simulink library "NCR18650BD_98S45P_Library"  (R2025a)
settings: Solver=VariableStepAuto  StartTime=0.0  StopTime=10.0  RelTol=1e-3
undefined symbols (not defined in the file or in its folder): battery_builder_rtmsupport, gcbh
libraries: NCR18650BD_98S45P_Library_lib x16
(part 1 of 2)
settings Model: Creator=saarv  LastModifiedBy=saarv

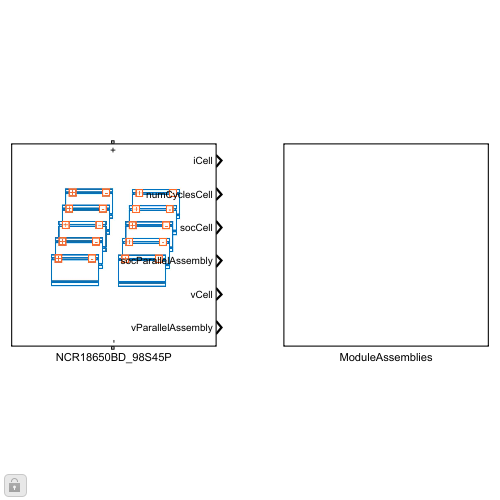
[thumbnail: Simulink's stored preview of the top-level diagram]
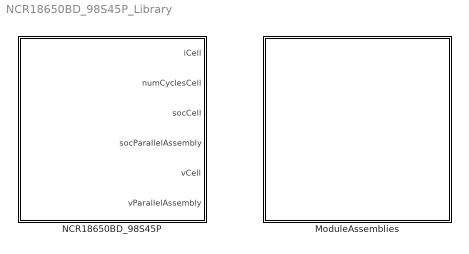
== system NCR18650BD_98S45P_Library ==
  ModuleAssemblies : Subsystem
  NCR18650BD_98S45P : Subsystem  LoadFcn=battery_builder_rtmsupport('loadfcn',gcbh);
      settings: CopyFcn=battery_builder_rtmsupport('copyfcn',gcbh);  PreCopyFcn=battery_builder_rtmsupport('precopyfcn',gcbh);  PreDeleteFcn=battery_builder_rtmsupport('predeletefcn',gcbh);  PortSchema="{\"entries\":[{\"content\":{\"sides\":[{\"content\":{\"connectorIds\":[\"LConn1\"]},\"type\":\"ConnectorPlacement.EquallySpacedRectSide\",\"uuid\":\"9e7041d5-d3d9-4996-bd95-b169094aaa75\"},{\"content\":{\"connectorIds\":[\"RConn1\"],\"side\":\"RIGHT\"},\"type\":\"ConnectorPlacement.EquallySpacedRectSide\",\"uuid\":\"1a9d726b-e110-445d-9094-f9af8985733a\"},{\"content\":{\"side\":\"TOP\"},\"type\":\"ConnectorPlacement.EquallySpacedRectSide\",\"uuid\":\"c9094138-05f6-46bf-9d7c-2f9307e18b10\"},{\"content\":{\"connectorIds\":[\"Out1\",\"Out2\",\"Out3\",\"Out4\",\"Out5\",\"Out6\"],\"side\":\"BOTTOM\"},\"type\":\"ConnectorPlacement.EquallySpacedRectSide\",\"uuid\":\"12959d5d-2702-4b18-986c-5ba3b231edc9\"}]},\"type\":\"ConnectorPlacement.EquallySpacedConnector\",\"uuid\":\"b4792a63-91de-4aa8-9329-1ac229a09e41\"}],\"packageUris\":[\"http://schema.mathworks.com/mf0/Connector/R2020b\"],\"version\":\"1.0\"}"
      mask Display: image('$imagefile')

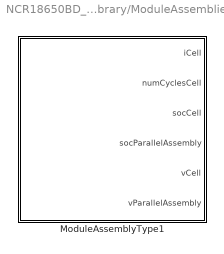
== system NCR18650BD_98S45P_Library/ModuleAssemblies ==
  ModuleAssemblyType1 : Subsystem  LoadFcn=battery_builder_rtmsupport('loadfcn',gcbh);
      settings: CopyFcn=battery_builder_rtmsupport('copyfcn',gcbh);  PreCopyFcn=battery_builder_rtmsupport('precopyfcn',gcbh);  PreDeleteFcn=battery_builder_rtmsupport('predeletefcn',gcbh);  PortSchema="{\"entries\":[{\"content\":{\"sides\":[{\"content\":{\"connectorIds\":[\"LConn1\"]},\"type\":\"ConnectorPlacement.EquallySpacedRectSide\",\"uuid\":\"9e7041d5-d3d9-4996-bd95-b169094aaa75\"},{\"content\":{\"connectorIds\":[\"RConn1\"],\"side\":\"RIGHT\"},\"type\":\"ConnectorPlacement.EquallySpacedRectSide\",\"uuid\":\"1a9d726b-e110-445d-9094-f9af8985733a\"},{\"content\":{\"side\":\"TOP\"},\"type\":\"ConnectorPlacement.EquallySpacedRectSide\",\"uuid\":\"c9094138-05f6-46bf-9d7c-2f9307e18b10\"},{\"content\":{\"connectorIds\":[\"Out1\",\"Out2\",\"Out3\",\"Out4\",\"Out5\",\"Out6\"],\"side\":\"BOTTOM\"},\"type\":\"ConnectorPlacement.EquallySpacedRectSide\",\"uuid\":\"a73cbc57-fefd-438e-a02a-7299c4782ae8\"}]},\"type\":\"ConnectorPlacement.EquallySpacedConnector\",\"uuid\":\"b4792a63-91de-4aa8-9329-1ac229a09e41\"}],\"packageUris\":[\"http://schema.mathworks.com/mf0/Connector/R2020b\"],\"version\":\"1.0\"}"
      mask Display: image('$imagefile')

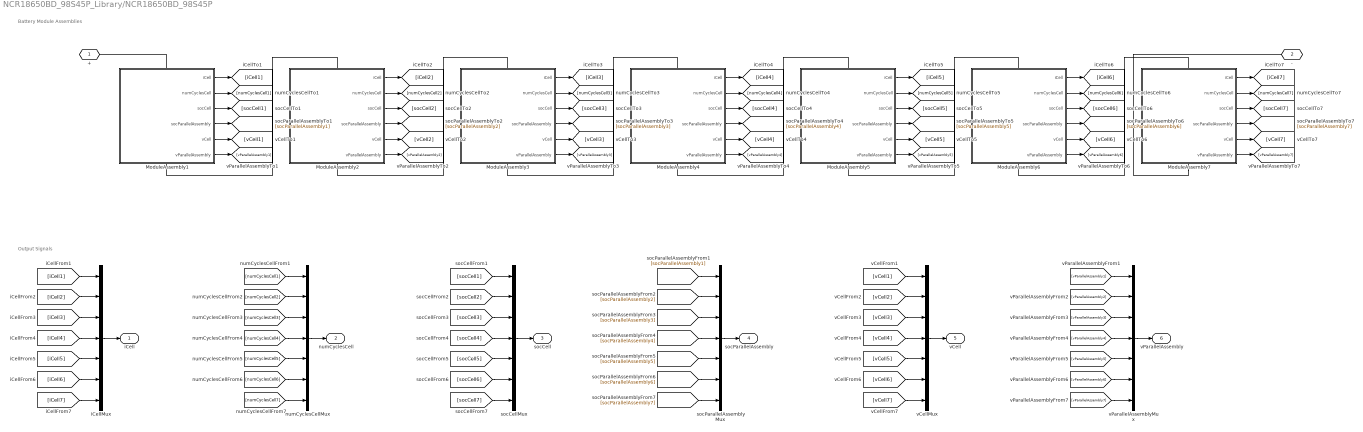
== system NCR18650BD_98S45P_Library/NCR18650BD_98S45P ==
  note: Battery Module Assemblies
  note: Output Signals
  ModuleAssembly1 : Subsystem  LoadFcn=battery_builder_rtmsupport('loadfcn',gcbh);
      settings: CopyFcn=battery_builder_rtmsupport('copyfcn',gcbh);  PreCopyFcn=battery_builder_rtmsupport('precopyfcn',gcbh);  PreDeleteFcn=battery_builder_rtmsupport('predeletefcn',gcbh);  PortSchema="{\"entries\":[{\"content\":{\"sides\":[{\"content\":{\"connectorIds\":[\"LConn1\"]},\"type\":\"ConnectorPlacement.EquallySpacedRectSide\",\"uuid\":\"9e7041d5-d3d9-4996-bd95-b169094aaa75\"},{\"content\":{\"connectorIds\":[\"RConn1\"],\"side\":\"RIGHT\"},\"type\":\"ConnectorPlacement.EquallySpacedRectSide\",\"uuid\":\"1a9d726b-e110-445d-9094-f9af8985733a\"},{\"content\":{\"side\":\"TOP\"},\"type\":\"ConnectorPlacement.EquallySpacedRectSide\",\"uuid\":\"c9094138-05f6-46bf-9d7c-2f9307e18b10\"},{\"content\":{\"connectorIds\":[\"Out1\",\"Out2\",\"Out3\",\"Out4\",\"Out5\",\"Out6\"],\"side\":\"BOTTOM\"},\"type\":\"ConnectorPlacement.EquallySpacedRectSide\",\"uuid\":\"a73cbc57-fefd-438e-a02a-7299c4782ae8\"}]},\"type\":\"ConnectorPlacement.EquallySpacedConnector\",\"uuid\":\"b4792a63-91de-4aa8-9329-1ac229a09e41\"}],\"packageUris\":[\"http://schema.mathworks.com/mf0/Connector/R2020b\"],\"version\":\"1.0\"}"
      mask Display: image('$imagefile')
  ModuleAssembly2 : Subsystem  LoadFcn=battery_builder_rtmsupport('loadfcn',gcbh);
      settings: CopyFcn=battery_builder_rtmsupport('copyfcn',gcbh);  PreCopyFcn=battery_builder_rtmsupport('precopyfcn',gcbh);  PreDeleteFcn=battery_builder_rtmsupport('predeletefcn',gcbh);  PortSchema="{\"entries\":[{\"content\":{\"sides\":[{\"content\":{\"connectorIds\":[\"LConn1\"]},\"type\":\"ConnectorPlacement.EquallySpacedRectSide\",\"uuid\":\"9e7041d5-d3d9-4996-bd95-b169094aaa75\"},{\"content\":{\"connectorIds\":[\"RConn1\"],\"side\":\"RIGHT\"},\"type\":\"ConnectorPlacement.EquallySpacedRectSide\",\"uuid\":\"1a9d726b-e110-445d-9094-f9af8985733a\"},{\"content\":{\"side\":\"TOP\"},\"type\":\"ConnectorPlacement.EquallySpacedRectSide\",\"uuid\":\"c9094138-05f6-46bf-9d7c-2f9307e18b10\"},{\"content\":{\"connectorIds\":[\"Out1\",\"Out2\",\"Out3\",\"Out4\",\"Out5\",\"Out6\"],\"side\":\"BOTTOM\"},\"type\":\"ConnectorPlacement.EquallySpacedRectSide\",\"uuid\":\"a73cbc57-fefd-438e-a02a-7299c4782ae8\"}]},\"type\":\"ConnectorPlacement.EquallySpacedConnector\",\"uuid\":\"b4792a63-91de-4aa8-9329-1ac229a09e41\"}],\"packageUris\":[\"http://schema.mathworks.com/mf0/Connector/R2020b\"],\"version\":\"1.0\"}"
      mask Display: image('$imagefile')
  ModuleAssembly3 : Subsystem  LoadFcn=battery_builder_rtmsupport('loadfcn',gcbh);
      settings: CopyFcn=battery_builder_rtmsupport('copyfcn',gcbh);  PreCopyFcn=battery_builder_rtmsupport('precopyfcn',gcbh);  PreDeleteFcn=battery_builder_rtmsupport('predeletefcn',gcbh);  PortSchema="{\"entries\":[{\"content\":{\"sides\":[{\"content\":{\"connectorIds\":[\"LConn1\"]},\"type\":\"ConnectorPlacement.EquallySpacedRectSide\",\"uuid\":\"9e7041d5-d3d9-4996-bd95-b169094aaa75\"},{\"content\":{\"connectorIds\":[\"RConn1\"],\"side\":\"RIGHT\"},\"type\":\"ConnectorPlacement.EquallySpacedRectSide\",\"uuid\":\"1a9d726b-e110-445d-9094-f9af8985733a\"},{\"content\":{\"side\":\"TOP\"},\"type\":\"ConnectorPlacement.EquallySpacedRectSide\",\"uuid\":\"c9094138-05f6-46bf-9d7c-2f9307e18b10\"},{\"content\":{\"connectorIds\":[\"Out1\",\"Out2\",\"Out3\",\"Out4\",\"Out5\",\"Out6\"],\"side\":\"BOTTOM\"},\"type\":\"ConnectorPlacement.EquallySpacedRectSide\",\"uuid\":\"a73cbc57-fefd-438e-a02a-7299c4782ae8\"}]},\"type\":\"ConnectorPlacement.EquallySpacedConnector\",\"uuid\":\"b4792a63-91de-4aa8-9329-1ac229a09e41\"}],\"packageUris\":[\"http://schema.mathworks.com/mf0/Connector/R2020b\"],\"version\":\"1.0\"}"
      mask Display: image('$imagefile')
  ModuleAssembly4 : Subsystem  LoadFcn=battery_builder_rtmsupport('loadfcn',gcbh);
      settings: CopyFcn=battery_builder_rtmsupport('copyfcn',gcbh);  PreCopyFcn=battery_builder_rtmsupport('precopyfcn',gcbh);  PreDeleteFcn=battery_builder_rtmsupport('predeletefcn',gcbh);  PortSchema="{\"entries\":[{\"content\":{\"sides\":[{\"content\":{\"connectorIds\":[\"LConn1\"]},\"type\":\"ConnectorPlacement.EquallySpacedRectSide\",\"uuid\":\"9e7041d5-d3d9-4996-bd95-b169094aaa75\"},{\"content\":{\"connectorIds\":[\"RConn1\"],\"side\":\"RIGHT\"},\"type\":\"ConnectorPlacement.EquallySpacedRectSide\",\"uuid\":\"1a9d726b-e110-445d-9094-f9af8985733a\"},{\"content\":{\"side\":\"TOP\"},\"type\":\"ConnectorPlacement.EquallySpacedRectSide\",\"uuid\":\"c9094138-05f6-46bf-9d7c-2f9307e18b10\"},{\"content\":{\"connectorIds\":[\"Out1\",\"Out2\",\"Out3\",\"Out4\",\"Out5\",\"Out6\"],\"side\":\"BOTTOM\"},\"type\":\"ConnectorPlacement.EquallySpacedRectSide\",\"uuid\":\"a73cbc57-fefd-438e-a02a-7299c4782ae8\"}]},\"type\":\"ConnectorPlacement.EquallySpacedConnector\",\"uuid\":\"b4792a63-91de-4aa8-9329-1ac229a09e41\"}],\"packageUris\":[\"http://schema.mathworks.com/mf0/Connector/R2020b\"],\"version\":\"1.0\"}"
      mask Display: image('$imagefile')
  ModuleAssembly5 : Subsystem  LoadFcn=battery_builder_rtmsupport('loadfcn',gcbh);
      settings: CopyFcn=battery_builder_rtmsupport('copyfcn',gcbh);  PreCopyFcn=battery_builder_rtmsupport('precopyfcn',gcbh);  PreDeleteFcn=battery_builder_rtmsupport('predeletefcn',gcbh);  PortSchema="{\"entries\":[{\"content\":{\"sides\":[{\"content\":{\"connectorIds\":[\"LConn1\"]},\"type\":\"ConnectorPlacement.EquallySpacedRectSide\",\"uuid\":\"9e7041d5-d3d9-4996-bd95-b169094aaa75\"},{\"content\":{\"connectorIds\":[\"RConn1\"],\"side\":\"RIGHT\"},\"type\":\"ConnectorPlacement.EquallySpacedRectSide\",\"uuid\":\"1a9d726b-e110-445d-9094-f9af8985733a\"},{\"content\":{\"side\":\"TOP\"},\"type\":\"ConnectorPlacement.EquallySpacedRectSide\",\"uuid\":\"c9094138-05f6-46bf-9d7c-2f9307e18b10\"},{\"content\":{\"connectorIds\":[\"Out1\",\"Out2\",\"Out3\",\"Out4\",\"Out5\",\"Out6\"],\"side\":\"BOTTOM\"},\"type\":\"ConnectorPlacement.EquallySpacedRectSide\",\"uuid\":\"a73cbc57-fefd-438e-a02a-7299c4782ae8\"}]},\"type\":\"ConnectorPlacement.EquallySpacedConnector\",\"uuid\":\"b4792a63-91de-4aa8-9329-1ac229a09e41\"}],\"packageUris\":[\"http://schema.mathworks.com/mf0/Connector/R2020b\"],\"version\":\"1.0\"}"
      mask Display: image('$imagefile')
  ModuleAssembly6 : Subsystem  LoadFcn=battery_builder_rtmsupport('loadfcn',gcbh);
      settings: CopyFcn=battery_builder_rtmsupport('copyfcn',gcbh);  PreCopyFcn=battery_builder_rtmsupport('precopyfcn',gcbh);  PreDeleteFcn=battery_builder_rtmsupport('predeletefcn',gcbh);  PortSchema="{\"entries\":[{\"content\":{\"sides\":[{\"content\":{\"connectorIds\":[\"LConn1\"]},\"type\":\"ConnectorPlacement.EquallySpacedRectSide\",\"uuid\":\"9e7041d5-d3d9-4996-bd95-b169094aaa75\"},{\"content\":{\"connectorIds\":[\"RConn1\"],\"side\":\"RIGHT\"},\"type\":\"ConnectorPlacement.EquallySpacedRectSide\",\"uuid\":\"1a9d726b-e110-445d-9094-f9af8985733a\"},{\"content\":{\"side\":\"TOP\"},\"type\":\"ConnectorPlacement.EquallySpacedRectSide\",\"uuid\":\"c9094138-05f6-46bf-9d7c-2f9307e18b10\"},{\"content\":{\"connectorIds\":[\"Out1\",\"Out2\",\"Out3\",\"Out4\",\"Out5\",\"Out6\"],\"side\":\"BOTTOM\"},\"type\":\"ConnectorPlacement.EquallySpacedRectSide\",\"uuid\":\"a73cbc57-fefd-438e-a02a-7299c4782ae8\"}]},\"type\":\"ConnectorPlacement.EquallySpacedConnector\",\"uuid\":\"b4792a63-91de-4aa8-9329-1ac229a09e41\"}],\"packageUris\":[\"http://schema.mathworks.com/mf0/Connector/R2020b\"],\"version\":\"1.0\"}"
      mask Display: image('$imagefile')
  ModuleAssembly7 : Subsystem  LoadFcn=battery_builder_rtmsupport('loadfcn',gcbh);
      settings: CopyFcn=battery_builder_rtmsupport('copyfcn',gcbh);  PreCopyFcn=battery_builder_rtmsupport('precopyfcn',gcbh);  PreDeleteFcn=battery_builder_rtmsupport('predeletefcn',gcbh);  PortSchema="{\"entries\":[{\"content\":{\"sides\":[{\"content\":{\"connectorIds\":[\"LConn1\"]},\"type\":\"ConnectorPlacement.EquallySpacedRectSide\",\"uuid\":\"9e7041d5-d3d9-4996-bd95-b169094aaa75\"},{\"content\":{\"connectorIds\":[\"RConn1\"],\"side\":\"RIGHT\"},\"type\":\"ConnectorPlacement.EquallySpacedRectSide\",\"uuid\":\"1a9d726b-e110-445d-9094-f9af8985733a\"},{\"content\":{\"side\":\"TOP\"},\"type\":\"ConnectorPlacement.EquallySpacedRectSide\",\"uuid\":\"c9094138-05f6-46bf-9d7c-2f9307e18b10\"},{\"content\":{\"connectorIds\":[\"Out1\",\"Out2\",\"Out3\",\"Out4\",\"Out5\",\"Out6\"],\"side\":\"BOTTOM\"},\"type\":\"ConnectorPlacement.EquallySpacedRectSide\",\"uuid\":\"a73cbc57-fefd-438e-a02a-7299c4782ae8\"}]},\"type\":\"ConnectorPlacement.EquallySpacedConnector\",\"uuid\":\"b4792a63-91de-4aa8-9329-1ac229a09e41\"}],\"packageUris\":[\"http://schema.mathworks.com/mf0/Connector/R2020b\"],\"version\":\"1.0\"}"
      mask Display: image('$imagefile')
  iCellMux : Mux  Inputs=7
  numCyclesCellMux : Mux  Inputs=7
  socCellMux : Mux  Inputs=7
  socParallelAssemblyMux : Mux  Inputs=7
  vCellMux : Mux  Inputs=7
  vParallelAssemblyMux : Mux  Inputs=7
  + : PMIOPort  Side=Left
  - : PMIOPort  Port=2  Side=Right
  iCell : Outport
  numCyclesCell : Outport  Port=2
  socCell : Outport  Port=3
  socParallelAssembly : Outport  Port=4
  vCell : Outport  Port=5
  vParallelAssembly : Outport  Port=6
  wires:
  ModuleAssembly1/1(iCell) -> [iCell1]
  iCellMux/1 -> iCell/1
  [iCell1] -> iCellMux/1
  ModuleAssembly1/2(numCyclesCell) -> [numCyclesCell1]
  numCyclesCellMux/1 -> numCyclesCell/1
  [numCyclesCell1] -> numCyclesCellMux/1
  ModuleAssembly1/3(socCell) -> [socCell1]
  socCellMux/1 -> socCell/1
  [socCell1] -> socCellMux/1
  ModuleAssembly1/4(socParallelAssembly) -> [socParallelAssembly1]
  socParallelAssemblyMux/1 -> socParallelAssembly/1
  [socParallelAssembly1] -> socParallelAssemblyMux/1
  ModuleAssembly1/5(vCell) -> [vCell1]
  vCellMux/1 -> vCell/1
  [vCell1] -> vCellMux/1
  ModuleAssembly1/6(vParallelAssembly) -> [vParallelAssembly1]
  vParallelAssemblyMux/1 -> vParallelAssembly/1
  [vParallelAssembly1] -> vParallelAssemblyMux/1
  ModuleAssembly2/1(iCell) -> [iCell2]
  [iCell2] -> iCellMux/2
  ModuleAssembly2/2(numCyclesCell) -> [numCyclesCell2]
  [numCyclesCell2] -> numCyclesCellMux/2
  ModuleAssembly2/3(socCell) -> [socCell2]
  [socCell2] -> socCellMux/2
  ModuleAssembly2/4(socParallelAssembly) -> [socParallelAssembly2]
  [socParallelAssembly2] -> socParallelAssemblyMux/2
  ModuleAssembly2/5(vCell) -> [vCell2]
  [vCell2] -> vCellMux/2
  ModuleAssembly2/6(vParallelAssembly) -> [vParallelAssembly2]
  [vParallelAssembly2] -> vParallelAssemblyMux/2
  ModuleAssembly3/1(iCell) -> [iCell3]
  [iCell3] -> iCellMux/3
  ModuleAssembly3/2(numCyclesCell) -> [numCyclesCell3]
  [numCyclesCell3] -> numCyclesCellMux/3
  ModuleAssembly3/3(socCell) -> [socCell3]
  [socCell3] -> socCellMux/3
  ModuleAssembly3/4(socParallelAssembly) -> [socParallelAssembly3]
  [socParallelAssembly3] -> socParallelAssemblyMux/3
  ModuleAssembly3/5(vCell) -> [vCell3]
  [vCell3] -> vCellMux/3
  ModuleAssembly3/6(vParallelAssembly) -> [vParallelAssembly3]
  [vParallelAssembly3] -> vParallelAssemblyMux/3
  ModuleAssembly4/1(iCell) -> [iCell4]
  [iCell4] -> iCellMux/4
  ModuleAssembly4/2(numCyclesCell) -> [numCyclesCell4]
  [numCyclesCell4] -> numCyclesCellMux/4
  ModuleAssembly4/3(socCell) -> [socCell4]
  [socCell4] -> socCellMux/4
  ModuleAssembly4/4(socParallelAssembly) -> [socParallelAssembly4]
  [socParallelAssembly4] -> socParallelAssemblyMux/4
  ModuleAssembly4/5(vCell) -> [vCell4]
  [vCell4] -> vCellMux/4
  ModuleAssembly4/6(vParallelAssembly) -> [vParallelAssembly4]
  [vParallelAssembly4] -> vParallelAssemblyMux/4
  ModuleAssembly5/1(iCell) -> [iCell5]
  [iCell5] -> iCellMux/5
  ModuleAssembly5/2(numCyclesCell) -> [numCyclesCell5]
  [numCyclesCell5] -> numCyclesCellMux/5
  ModuleAssembly5/3(socCell) -> [socCell5]
  [socCell5] -> socCellMux/5
  ModuleAssembly5/4(socParallelAssembly) -> [socParallelAssembly5]
  [socParallelAssembly5] -> socParallelAssemblyMux/5
  ModuleAssembly5/5(vCell) -> [vCell5]
  [vCell5] -> vCellMux/5
  ModuleAssembly5/6(vParallelAssembly) -> [vParallelAssembly5]
  [vParallelAssembly5] -> vParallelAssemblyMux/5
  ModuleAssembly6/1(iCell) -> [iCell6]
  [iCell6] -> iCellMux/6
  ModuleAssembly6/2(numCyclesCell) -> [numCyclesCell6]
  [numCyclesCell6] -> numCyclesCellMux/6
  ModuleAssembly6/3(socCell) -> [socCell6]
  [socCell6] -> socCellMux/6
  ModuleAssembly6/4(socParallelAssembly) -> [socParallelAssembly6]
  [socParallelAssembly6] -> socParallelAssemblyMux/6
  ModuleAssembly6/5(vCell) -> [vCell6]
  [vCell6] -> vCellMux/6
  ModuleAssembly6/6(vParallelAssembly) -> [vParallelAssembly6]
  [vParallelAssembly6] -> vParallelAssemblyMux/6
  ModuleAssembly7/1(iCell) -> [iCell7]
  [iCell7] -> iCellMux/7
  ModuleAssembly7/2(numCyclesCell) -> [numCyclesCell7]
  [numCyclesCell7] -> numCyclesCellMux/7
  ModuleAssembly7/3(socCell) -> [socCell7]
  [socCell7] -> socCellMux/7
  ModuleAssembly7/4(socParallelAssembly) -> [socParallelAssembly7]
  [socParallelAssembly7] -> socParallelAssemblyMux/7
  ModuleAssembly7/5(vCell) -> [vCell7]
  [vCell7] -> vCellMux/7
  ModuleAssembly7/6(vParallelAssembly) -> [vParallelAssembly7]
  [vParallelAssembly7] -> vParallelAssemblyMux/7
  connections:
  ModuleAssembly2/LConn1 -- ModuleAssembly1/RConn1
  ModuleAssembly3/LConn1 -- ModuleAssembly2/RConn1
  ModuleAssembly4/LConn1 -- ModuleAssembly3/RConn1
  ModuleAssembly5/LConn1 -- ModuleAssembly4/RConn1
  ModuleAssembly6/LConn1 -- ModuleAssembly5/RConn1
  ModuleAssembly7/LConn1 -- ModuleAssembly6/RConn1
  ModuleAssembly1/LConn1 -- +/RConn1
  ModuleAssembly7/RConn1 -- -/RConn1

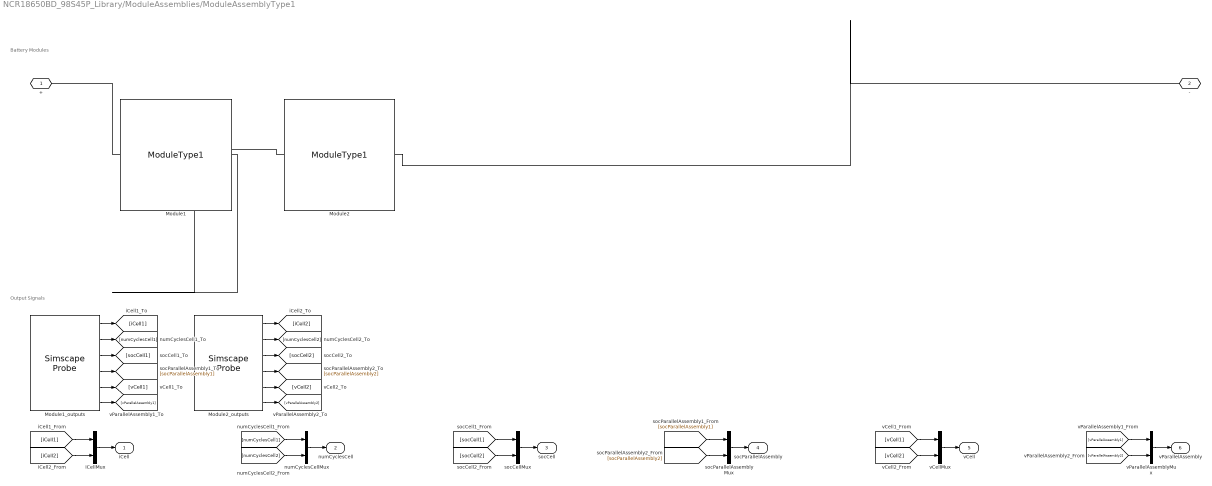
== system NCR18650BD_98S45P_Library/ModuleAssemblies/ModuleAssemblyType1 ==
  note: Battery Modules
  note: Output Signals
  Module1 : NCR18650BD_98S45P_Library_lib/Modules/ModuleType1  SOC_vecCell=[0, .1, .25, .5, .75, .9, 1]  V0_vecCell=[3.5057, 3.566, 3.6337, 3.7127, 3.9259, 4.0777, 4.1928] V  V_rangeCell=[0, inf] V  R0_vecCell=[.0085, .0085, .0087, .0082, .0083, .0085, .0085] Ohm  AHCell=27 A*hr  extrapolation_optionCell=simscape.enum.extrapolation.nearest  P=45  S=7  iCell_specify=off  iCell_priority=None  iCell=0 A  iCell_nominal_specify=off  iCell_nominal_value=1  iCell_nominal_unit=A  vCell_specify=off  vCell_priority=None  vCell=0 V  vCell_nominal_specify=off  vCell_nominal_value=1  vCell_nominal_unit=V  socCell_specify=off  socCell_priority=High  socCell=1  socCell_nominal_specify=off  socCell_nominal_value=1  socCell_nominal_unit=1  numCyclesCell_specify=off  numCyclesCell_priority=High  numCyclesCell=0  numCyclesCell_nominal_specify=off  numCyclesCell_nominal_value=1  numCyclesCell_nominal_unit=1  vParallelAssembly_specify=off  vParallelAssembly_priority=None  vParallelAssembly=repmat(0, 7, 1) V  vParallelAssembly_nominal_specify=off  vParallelAssembly_nominal_value=1  vParallelAssembly_nominal_unit=V  socParallelAssembly_specify=off  socParallelAssembly_priority=None  socParallelAssembly=repmat(1, 7, 1)  socParallelAssembly_nominal_specify=off  socParallelAssembly_nominal_value=1  socParallelAssembly_nominal_unit=1
      settings: InternalSimscapePortConfiguration="{\"Bottom\":[{\"id\":\"n\",\"label\":\"-\",\"type\":\"foundation.electrical.electrical\"}],\"Left\":[],\"Right\":[],\"Top\":[{\"id\":\"p\",\"label\":\"+\",\"type\":\"foundation.electrical.electrical\"}]}"
  Module1_outputs : SimscapeProbe  BoundBlock=3  Variables="{\"iCell\":{\"Probing\":\"ON\"},\"numCyclesCell\":{\"Probing\":\"ON\"},\"socCell\":{\"Probing\":\"ON\"},\"socParallelAssembly\":{\"Probing\":\"ON\"},\"vCell\":{\"Probing\":\"ON\"},\"vParallelAssembly\":{\"Probing\":\"ON\"}}"
  Module2 : NCR18650BD_98S45P_Library_lib/Modules/ModuleType1  SOC_vecCell=[0, .1, .25, .5, .75, .9, 1]  V0_vecCell=[3.5057, 3.566, 3.6337, 3.7127, 3.9259, 4.0777, 4.1928] V  V_rangeCell=[0, inf] V  R0_vecCell=[.0085, .0085, .0087, .0082, .0083, .0085, .0085] Ohm  AHCell=27 A*hr  extrapolation_optionCell=simscape.enum.extrapolation.nearest  P=45  S=7  iCell_specify=off  iCell_priority=None  iCell=0 A  iCell_nominal_specify=off  iCell_nominal_value=1  iCell_nominal_unit=A  vCell_specify=off  vCell_priority=None  vCell=0 V  vCell_nominal_specify=off  vCell_nominal_value=1  vCell_nominal_unit=V  socCell_specify=off  socCell_priority=High  socCell=1  socCell_nominal_specify=off  socCell_nominal_value=1  socCell_nominal_unit=1  numCyclesCell_specify=off  numCyclesCell_priority=High  numCyclesCell=0  numCyclesCell_nominal_specify=off  numCyclesCell_nominal_value=1  numCyclesCell_nominal_unit=1  vParallelAssembly_specify=off  vParallelAssembly_priority=None  vParallelAssembly=repmat(0, 7, 1) V  vParallelAssembly_nominal_specify=off  vParallelAssembly_nominal_value=1  vParallelAssembly_nominal_unit=V  socParallelAssembly_specify=off  socParallelAssembly_priority=None  socParallelAssembly=repmat(1, 7, 1)  socParallelAssembly_nominal_specify=off  socParallelAssembly_nominal_value=1  socParallelAssembly_nominal_unit=1
      settings: InternalSimscapePortConfiguration="{\"Bottom\":[{\"id\":\"n\",\"label\":\"-\",\"type\":\"foundation.electrical.electrical\"}],\"Left\":[],\"Right\":[],\"Top\":[{\"id\":\"p\",\"label\":\"+\",\"type\":\"foundation.electrical.electrical\"}]}"
  Module2_outputs : SimscapeProbe  BoundBlock=4  Variables="{\"iCell\":{\"Probing\":\"ON\"},\"numCyclesCell\":{\"Probing\":\"ON\"},\"socCell\":{\"Probing\":\"ON\"},\"socParallelAssembly\":{\"Probing\":\"ON\"},\"vCell\":{\"Probing\":\"ON\"},\"vParallelAssembly\":{\"Probing\":\"ON\"}}"
  iCellMux : Mux  Inputs=2
  numCyclesCellMux : Mux  Inputs=2
  socCellMux : Mux  Inputs=2
  socParallelAssemblyMux : Mux  Inputs=2
  vCellMux : Mux  Inputs=2
  vParallelAssemblyMux : Mux  Inputs=2
  + : PMIOPort  Side=Left
  - : PMIOPort  Port=2  Side=Right
  iCell : Outport
  numCyclesCell : Outport  Port=2
  socCell : Outport  Port=3
  socParallelAssembly : Outport  Port=4
  vCell : Outport  Port=5
  vParallelAssembly : Outport  Port=6
  wires:
  Module1_outputs/1 -> [iCell1]
  iCellMux/1 -> iCell/1
  [iCell1] -> iCellMux/1
  Module1_outputs/2 -> [numCyclesCell1]
  numCyclesCellMux/1 -> numCyclesCell/1
  [numCyclesCell1] -> numCyclesCellMux/1
  Module1_outputs/3 -> [socCell1]
  socCellMux/1 -> socCell/1
  [socCell1] -> socCellMux/1
  Module1_outputs/4 -> [socParallelAssembly1]
  socParallelAssemblyMux/1 -> socParallelAssembly/1
  [socParallelAssembly1] -> socParallelAssemblyMux/1
  Module1_outputs/5 -> [vCell1]
  vCellMux/1 -> vCell/1
  [vCell1] -> vCellMux/1
  Module1_outputs/6 -> [vParallelAssembly1]
  vParallelAssemblyMux/1 -> vParallelAssembly/1
  [vParallelAssembly1] -> vParallelAssemblyMux/1
  Module2_outputs/1 -> [iCell2]
  [iCell2] -> iCellMux/2
  Module2_outputs/2 -> [numCyclesCell2]
  [numCyclesCell2] -> numCyclesCellMux/2
  Module2_outputs/3 -> [socCell2]
  [socCell2] -> socCellMux/2
  Module2_outputs/4 -> [socParallelAssembly2]
  [socParallelAssembly2] -> socParallelAssemblyMux/2
  Module2_outputs/5 -> [vCell2]
  [vCell2] -> vCellMux/2
  Module2_outputs/6 -> [vParallelAssembly2]
  [vParallelAssembly2] -> vParallelAssemblyMux/2
  connections:
  Module2/LConn1 -- Module1/RConn1
  Module1/LConn1 -- +/RConn1
  Module2/RConn1 -- -/RConn1

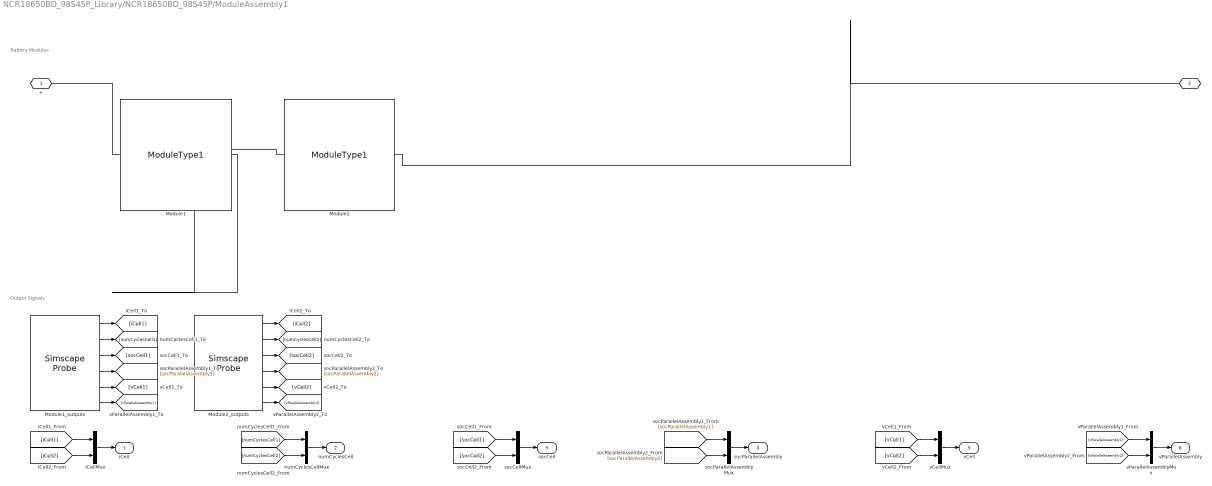
== system NCR18650BD_98S45P_Library/NCR18650BD_98S45P/ModuleAssembly1 ==
  note: Output Signals
  note: Battery Modules
  Module1 : NCR18650BD_98S45P_Library_lib/Modules/ModuleType1  SOC_vecCell=[0, .1, .25, .5, .75, .9, 1]  V0_vecCell=[3.5057, 3.566, 3.6337, 3.7127, 3.9259, 4.0777, 4.1928] V  V_rangeCell=[0, inf] V  R0_vecCell=[.0085, .0085, .0087, .0082, .0083, .0085, .0085] Ohm  AHCell=27 A*hr  extrapolation_optionCell=simscape.enum.extrapolation.nearest  P=45  S=7  iCell_specify=off  iCell_priority=None  iCell=0 A  iCell_nominal_specify=off  iCell_nominal_value=1  iCell_nominal_unit=A  vCell_specify=off  vCell_priority=None  vCell=0 V  vCell_nominal_specify=off  vCell_nominal_value=1  vCell_nominal_unit=V  socCell_specify=off  socCell_priority=High  socCell=1  socCell_nominal_specify=off  socCell_nominal_value=1  socCell_nominal_unit=1  numCyclesCell_specify=off  numCyclesCell_priority=High  numCyclesCell=0  numCyclesCell_nominal_specify=off  numCyclesCell_nominal_value=1  numCyclesCell_nominal_unit=1  vParallelAssembly_specify=off  vParallelAssembly_priority=None  vParallelAssembly=repmat(0, 7, 1) V  vParallelAssembly_nominal_specify=off  vParallelAssembly_nominal_value=1  vParallelAssembly_nominal_unit=V  socParallelAssembly_specify=off  socParallelAssembly_priority=None  socParallelAssembly=repmat(1, 7, 1)  socParallelAssembly_nominal_specify=off  socParallelAssembly_nominal_value=1  socParallelAssembly_nominal_unit=1
      settings: InternalSimscapePortConfiguration="{\"Bottom\":[{\"id\":\"n\",\"label\":\"-\",\"type\":\"foundation.electrical.electrical\"}],\"Left\":[],\"Right\":[],\"Top\":[{\"id\":\"p\",\"label\":\"+\",\"type\":\"foundation.electrical.electrical\"}]}"
  Module1_outputs : SimscapeProbe  BoundBlock=49  Variables="{\"iCell\":{\"Probing\":\"ON\"},\"numCyclesCell\":{\"Probing\":\"ON\"},\"socCell\":{\"Probing\":\"ON\"},\"socParallelAssembly\":{\"Probing\":\"ON\"},\"vCell\":{\"Probing\":\"ON\"},\"vParallelAssembly\":{\"Probing\":\"ON\"}}"
  Module2 : NCR18650BD_98S45P_Library_lib/Modules/ModuleType1  SOC_vecCell=[0, .1, .25, .5, .75, .9, 1]  V0_vecCell=[3.5057, 3.566, 3.6337, 3.7127, 3.9259, 4.0777, 4.1928] V  V_rangeCell=[0, inf] V  R0_vecCell=[.0085, .0085, .0087, .0082, .0083, .0085, .0085] Ohm  AHCell=27 A*hr  extrapolation_optionCell=simscape.enum.extrapolation.nearest  P=45  S=7  iCell_specify=off  iCell_priority=None  iCell=0 A  iCell_nominal_specify=off  iCell_nominal_value=1  iCell_nominal_unit=A  vCell_specify=off  vCell_priority=None  vCell=0 V  vCell_nominal_specify=off  vCell_nominal_value=1  vCell_nominal_unit=V  socCell_specify=off  socCell_priority=High  socCell=1  socCell_nominal_specify=off  socCell_nominal_value=1  socCell_nominal_unit=1  numCyclesCell_specify=off  numCyclesCell_priority=High  numCyclesCell=0  numCyclesCell_nominal_specify=off  numCyclesCell_nominal_value=1  numCyclesCell_nominal_unit=1  vParallelAssembly_specify=off  vParallelAssembly_priority=None  vParallelAssembly=repmat(0, 7, 1) V  vParallelAssembly_nominal_specify=off  vParallelAssembly_nominal_value=1  vParallelAssembly_nominal_unit=V  socParallelAssembly_specify=off  socParallelAssembly_priority=None  socParallelAssembly=repmat(1, 7, 1)  socParallelAssembly_nominal_specify=off  socParallelAssembly_nominal_value=1  socParallelAssembly_nominal_unit=1
      settings: InternalSimscapePortConfiguration="{\"Bottom\":[{\"id\":\"n\",\"label\":\"-\",\"type\":\"foundation.electrical.electrical\"}],\"Left\":[],\"Right\":[],\"Top\":[{\"id\":\"p\",\"label\":\"+\",\"type\":\"foundation.electrical.electrical\"}]}"
  Module2_outputs : SimscapeProbe  BoundBlock=51  Variables="{\"iCell\":{\"Probing\":\"ON\"},\"numCyclesCell\":{\"Probing\":\"ON\"},\"socCell\":{\"Probing\":\"ON\"},\"socParallelAssembly\":{\"Probing\":\"ON\"},\"vCell\":{\"Probing\":\"ON\"},\"vParallelAssembly\":{\"Probing\":\"ON\"}}"
  iCellMux : Mux  Inputs=2
  numCyclesCellMux : Mux  Inputs=2
  socCellMux : Mux  Inputs=2
  socParallelAssemblyMux : Mux  Inputs=2
  vCellMux : Mux  Inputs=2
  vParallelAssemblyMux : Mux  Inputs=2
  + : PMIOPort  Side=Left
  - : PMIOPort  Port=2  Side=Right
  iCell : Outport
  numCyclesCell : Outport  Port=2
  socCell : Outport  Port=3
  socParallelAssembly : Outport  Port=4
  vCell : Outport  Port=5
  vParallelAssembly : Outport  Port=6
  wires:
  [vParallelAssembly2] -> vParallelAssemblyMux/2
  Module2_outputs/6 -> [vParallelAssembly2]
  [vCell2] -> vCellMux/2
  Module2_outputs/5 -> [vCell2]
  [socParallelAssembly2] -> socParallelAssemblyMux/2
  Module2_outputs/4 -> [socParallelAssembly2]
  [socCell2] -> socCellMux/2
  Module2_outputs/3 -> [socCell2]
  [numCyclesCell2] -> numCyclesCellMux/2
  Module2_outputs/2 -> [numCyclesCell2]
  [iCell2] -> iCellMux/2
  Module2_outputs/1 -> [iCell2]
  [vParallelAssembly1] -> vParallelAssemblyMux/1
  vParallelAssemblyMux/1 -> vParallelAssembly/1
  Module1_outputs/6 -> [vParallelAssembly1]
  [vCell1] -> vCellMux/1
  vCellMux/1 -> vCell/1
  Module1_outputs/5 -> [vCell1]
  [socParallelAssembly1] -> socParallelAssemblyMux/1
  socParallelAssemblyMux/1 -> socParallelAssembly/1
  Module1_outputs/4 -> [socParallelAssembly1]
  [socCell1] -> socCellMux/1
  socCellMux/1 -> socCell/1
  Module1_outputs/3 -> [socCell1]
  [numCyclesCell1] -> numCyclesCellMux/1
  numCyclesCellMux/1 -> numCyclesCell/1
  Module1_outputs/2 -> [numCyclesCell1]
  [iCell1] -> iCellMux/1
  iCellMux/1 -> iCell/1
  Module1_outputs/1 -> [iCell1]
  connections:
  Module2/RConn1 -- -/RConn1
  Module1/LConn1 -- +/RConn1
  Module2/LConn1 -- Module1/RConn1

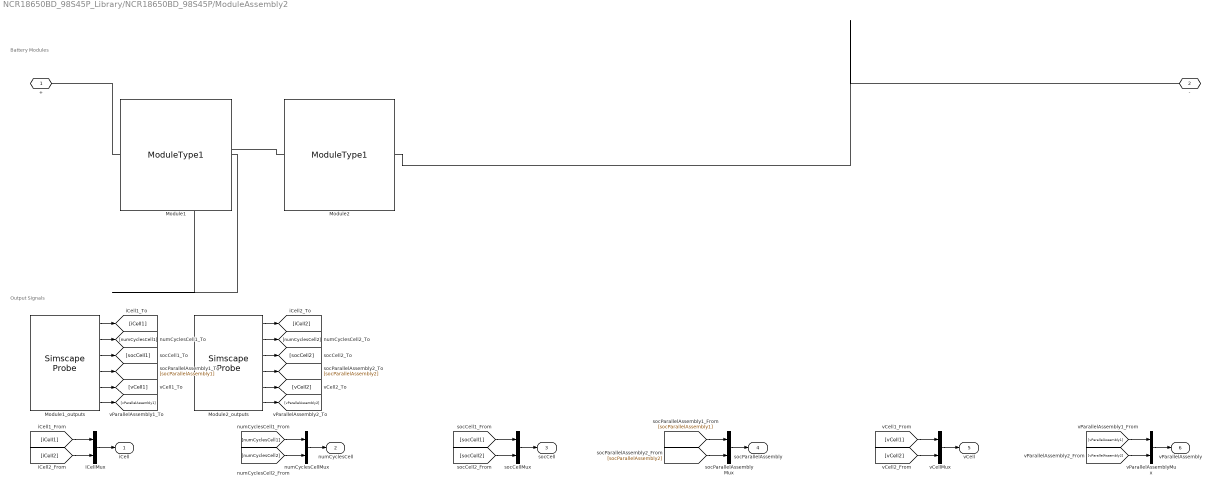
== system NCR18650BD_98S45P_Library/NCR18650BD_98S45P/ModuleAssembly2 ==
  note: Output Signals
  note: Battery Modules
  Module1 : NCR18650BD_98S45P_Library_lib/Modules/ModuleType1  SOC_vecCell=[0, .1, .25, .5, .75, .9, 1]  V0_vecCell=[3.5057, 3.566, 3.6337, 3.7127, 3.9259, 4.0777, 4.1928] V  V_rangeCell=[0, inf] V  R0_vecCell=[.0085, .0085, .0087, .0082, .0083, .0085, .0085] Ohm  AHCell=27 A*hr  extrapolation_optionCell=simscape.enum.extrapolation.nearest  P=45  S=7  iCell_specify=off  iCell_priority=None  iCell=0 A  iCell_nominal_specify=off  iCell_nominal_value=1  iCell_nominal_unit=A  vCell_specify=off  vCell_priority=None  vCell=0 V  vCell_nominal_specify=off  vCell_nominal_value=1  vCell_nominal_unit=V  socCell_specify=off  socCell_priority=High  socCell=1  socCell_nominal_specify=off  socCell_nominal_value=1  socCell_nominal_unit=1  numCyclesCell_specify=off  numCyclesCell_priority=High  numCyclesCell=0  numCyclesCell_nominal_specify=off  numCyclesCell_nominal_value=1  numCyclesCell_nominal_unit=1  vParallelAssembly_specify=off  vParallelAssembly_priority=None  vParallelAssembly=repmat(0, 7, 1) V  vParallelAssembly_nominal_specify=off  vParallelAssembly_nominal_value=1  vParallelAssembly_nominal_unit=V  socParallelAssembly_specify=off  socParallelAssembly_priority=None  socParallelAssembly=repmat(1, 7, 1)  socParallelAssembly_nominal_specify=off  socParallelAssembly_nominal_value=1  socParallelAssembly_nominal_unit=1
      settings: InternalSimscapePortConfiguration="{\"Bottom\":[{\"id\":\"n\",\"label\":\"-\",\"type\":\"foundation.electrical.electrical\"}],\"Left\":[],\"Right\":[],\"Top\":[{\"id\":\"p\",\"label\":\"+\",\"type\":\"foundation.electrical.electrical\"}]}"
  Module1_outputs : SimscapeProbe  BoundBlock=94  Variables="{\"iCell\":{\"Probing\":\"ON\"},\"numCyclesCell\":{\"Probing\":\"ON\"},\"socCell\":{\"Probing\":\"ON\"},\"socParallelAssembly\":{\"Probing\":\"ON\"},\"vCell\":{\"Probing\":\"ON\"},\"vParallelAssembly\":{\"Probing\":\"ON\"}}"
  Module2 : NCR18650BD_98S45P_Library_lib/Modules/ModuleType1  SOC_vecCell=[0, .1, .25, .5, .75, .9, 1]  V0_vecCell=[3.5057, 3.566, 3.6337, 3.7127, 3.9259, 4.0777, 4.1928] V  V_rangeCell=[0, inf] V  R0_vecCell=[.0085, .0085, .0087, .0082, .0083, .0085, .0085] Ohm  AHCell=27 A*hr  extrapolation_optionCell=simscape.enum.extrapolation.nearest  P=45  S=7  iCell_specify=off  iCell_priority=None  iCell=0 A  iCell_nominal_specify=off  iCell_nominal_value=1  iCell_nominal_unit=A  vCell_specify=off  vCell_priority=None  vCell=0 V  vCell_nominal_specify=off  vCell_nominal_value=1  vCell_nominal_unit=V  socCell_specify=off  socCell_priority=High  socCell=1  socCell_nominal_specify=off  socCell_nominal_value=1  socCell_nominal_unit=1  numCyclesCell_specify=off  numCyclesCell_priority=High  numCyclesCell=0  numCyclesCell_nominal_specify=off  numCyclesCell_nominal_value=1  numCyclesCell_nominal_unit=1  vParallelAssembly_specify=off  vParallelAssembly_priority=None  vParallelAssembly=repmat(0, 7, 1) V  vParallelAssembly_nominal_specify=off  vParallelAssembly_nominal_value=1  vParallelAssembly_nominal_unit=V  socParallelAssembly_specify=off  socParallelAssembly_priority=None  socParallelAssembly=repmat(1, 7, 1)  socParallelAssembly_nominal_specify=off  socParallelAssembly_nominal_value=1  socParallelAssembly_nominal_unit=1
      settings: InternalSimscapePortConfiguration="{\"Bottom\":[{\"id\":\"n\",\"label\":\"-\",\"type\":\"foundation.electrical.electrical\"}],\"Left\":[],\"Right\":[],\"Top\":[{\"id\":\"p\",\"label\":\"+\",\"type\":\"foundation.electrical.electrical\"}]}"
  Module2_outputs : SimscapeProbe  BoundBlock=96  Variables="{\"iCell\":{\"Probing\":\"ON\"},\"numCyclesCell\":{\"Probing\":\"ON\"},\"socCell\":{\"Probing\":\"ON\"},\"socParallelAssembly\":{\"Probing\":\"ON\"},\"vCell\":{\"Probing\":\"ON\"},\"vParallelAssembly\":{\"Probing\":\"ON\"}}"
  iCellMux : Mux  Inputs=2
  numCyclesCellMux : Mux  Inputs=2
  socCellMux : Mux  Inputs=2
  socParallelAssemblyMux : Mux  Inputs=2
  vCellMux : Mux  Inputs=2
  vParallelAssemblyMux : Mux  Inputs=2
  + : PMIOPort  Side=Left
  - : PMIOPort  Port=2  Side=Right
  iCell : Outport
  numCyclesCell : Outport  Port=2
  socCell : Outport  Port=3
  socParallelAssembly : Outport  Port=4
  vCell : Outport  Port=5
  vParallelAssembly : Outport  Port=6
  wires:
  [vParallelAssembly2] -> vParallelAssemblyMux/2
  Module2_outputs/6 -> [vParallelAssembly2]
  [vCell2] -> vCellMux/2
  Module2_outputs/5 -> [vCell2]
  [socParallelAssembly2] -> socParallelAssemblyMux/2
  Module2_outputs/4 -> [socParallelAssembly2]
  [socCell2] -> socCellMux/2
  Module2_outputs/3 -> [socCell2]
  [numCyclesCell2] -> numCyclesCellMux/2
  Module2_outputs/2 -> [numCyclesCell2]
  [iCell2] -> iCellMux/2
  Module2_outputs/1 -> [iCell2]
  [vParallelAssembly1] -> vParallelAssemblyMux/1
  vParallelAssemblyMux/1 -> vParallelAssembly/1
  Module1_outputs/6 -> [vParallelAssembly1]
  [vCell1] -> vCellMux/1
  vCellMux/1 -> vCell/1
  Module1_outputs/5 -> [vCell1]
  [socParallelAssembly1] -> socParallelAssemblyMux/1
  socParallelAssemblyMux/1 -> socParallelAssembly/1
  Module1_outputs/4 -> [socParallelAssembly1]
  [socCell1] -> socCellMux/1
  socCellMux/1 -> socCell/1
  Module1_outputs/3 -> [socCell1]
  [numCyclesCell1] -> numCyclesCellMux/1
  numCyclesCellMux/1 -> numCyclesCell/1
  Module1_outputs/2 -> [numCyclesCell1]
  [iCell1] -> iCellMux/1
  iCellMux/1 -> iCell/1
  Module1_outputs/1 -> [iCell1]
  connections:
  Module2/RConn1 -- -/RConn1
  Module1/LConn1 -- +/RConn1
  Module2/LConn1 -- Module1/RConn1

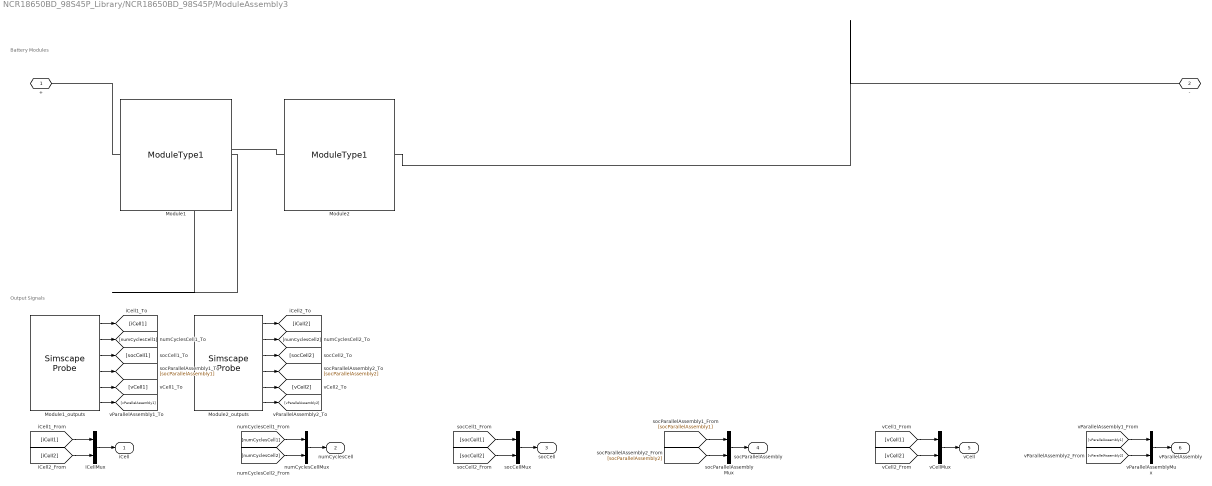
== system NCR18650BD_98S45P_Library/NCR18650BD_98S45P/ModuleAssembly3 ==
  note: Output Signals
  note: Battery Modules
  Module1 : NCR18650BD_98S45P_Library_lib/Modules/ModuleType1  SOC_vecCell=[0, .1, .25, .5, .75, .9, 1]  V0_vecCell=[3.5057, 3.566, 3.6337, 3.7127, 3.9259, 4.0777, 4.1928] V  V_rangeCell=[0, inf] V  R0_vecCell=[.0085, .0085, .0087, .0082, .0083, .0085, .0085] Ohm  AHCell=27 A*hr  extrapolation_optionCell=simscape.enum.extrapolation.nearest  P=45  S=7  iCell_specify=off  iCell_priority=None  iCell=0 A  iCell_nominal_specify=off  iCell_nominal_value=1  iCell_nominal_unit=A  vCell_specify=off  vCell_priority=None  vCell=0 V  vCell_nominal_specify=off  vCell_nominal_value=1  vCell_nominal_unit=V  socCell_specify=off  socCell_priority=High  socCell=1  socCell_nominal_specify=off  socCell_nominal_value=1  socCell_nominal_unit=1  numCyclesCell_specify=off  numCyclesCell_priority=High  numCyclesCell=0  numCyclesCell_nominal_specify=off  numCyclesCell_nominal_value=1  numCyclesCell_nominal_unit=1  vParallelAssembly_specify=off  vParallelAssembly_priority=None  vParallelAssembly=repmat(0, 7, 1) V  vParallelAssembly_nominal_specify=off  vParallelAssembly_nominal_value=1  vParallelAssembly_nominal_unit=V  socParallelAssembly_specify=off  socParallelAssembly_priority=None  socParallelAssembly=repmat(1, 7, 1)  socParallelAssembly_nominal_specify=off  socParallelAssembly_nominal_value=1  socParallelAssembly_nominal_unit=1
      settings: InternalSimscapePortConfiguration="{\"Bottom\":[{\"id\":\"n\",\"label\":\"-\",\"type\":\"foundation.electrical.electrical\"}],\"Left\":[],\"Right\":[],\"Top\":[{\"id\":\"p\",\"label\":\"+\",\"type\":\"foundation.electrical.electrical\"}]}"
  Module1_outputs : SimscapeProbe  BoundBlock=139  Variables="{\"iCell\":{\"Probing\":\"ON\"},\"numCyclesCell\":{\"Probing\":\"ON\"},\"socCell\":{\"Probing\":\"ON\"},\"socParallelAssembly\":{\"Probing\":\"ON\"},\"vCell\":{\"Probing\":\"ON\"},\"vParallelAssembly\":{\"Probing\":\"ON\"}}"
  Module2 : NCR18650BD_98S45P_Library_lib/Modules/ModuleType1  SOC_vecCell=[0, .1, .25, .5, .75, .9, 1]  V0_vecCell=[3.5057, 3.566, 3.6337, 3.7127, 3.9259, 4.0777, 4.1928] V  V_rangeCell=[0, inf] V  R0_vecCell=[.0085, .0085, .0087, .0082, .0083, .0085, .0085] Ohm  AHCell=27 A*hr  extrapolation_optionCell=simscape.enum.extrapolation.nearest  P=45  S=7  iCell_specify=off  iCell_priority=None  iCell=0 A  iCell_nominal_specify=off  iCell_nominal_value=1  iCell_nominal_unit=A  vCell_specify=off  vCell_priority=None  vCell=0 V  vCell_nominal_specify=off  vCell_nominal_value=1  vCell_nominal_unit=V  socCell_specify=off  socCell_priority=High  socCell=1  socCell_nominal_specify=off  socCell_nominal_value=1  socCell_nominal_unit=1  numCyclesCell_specify=off  numCyclesCell_priority=High  numCyclesCell=0  numCyclesCell_nominal_specify=off  numCyclesCell_nominal_value=1  numCyclesCell_nominal_unit=1  vParallelAssembly_specify=off  vParallelAssembly_priority=None  vParallelAssembly=repmat(0, 7, 1) V  vParallelAssembly_nominal_specify=off  vParallelAssembly_nominal_value=1  vParallelAssembly_nominal_unit=V  socParallelAssembly_specify=off  socParallelAssembly_priority=None  socParallelAssembly=repmat(1, 7, 1)  socParallelAssembly_nominal_specify=off  socParallelAssembly_nominal_value=1  socParallelAssembly_nominal_unit=1
      settings: InternalSimscapePortConfiguration="{\"Bottom\":[{\"id\":\"n\",\"label\":\"-\",\"type\":\"foundation.electrical.electrical\"}],\"Left\":[],\"Right\":[],\"Top\":[{\"id\":\"p\",\"label\":\"+\",\"type\":\"foundation.electrical.electrical\"}]}"
  Module2_outputs : SimscapeProbe  BoundBlock=141  Variables="{\"iCell\":{\"Probing\":\"ON\"},\"numCyclesCell\":{\"Probing\":\"ON\"},\"socCell\":{\"Probing\":\"ON\"},\"socParallelAssembly\":{\"Probing\":\"ON\"},\"vCell\":{\"Probing\":\"ON\"},\"vParallelAssembly\":{\"Probing\":\"ON\"}}"
  iCellMux : Mux  Inputs=2
  numCyclesCellMux : Mux  Inputs=2
  socCellMux : Mux  Inputs=2
  socParallelAssemblyMux : Mux  Inputs=2
  vCellMux : Mux  Inputs=2
  vParallelAssemblyMux : Mux  Inputs=2
  + : PMIOPort  Side=Left
  - : PMIOPort  Port=2  Side=Right
  iCell : Outport
  numCyclesCell : Outport  Port=2
  socCell : Outport  Port=3
  socParallelAssembly : Outport  Port=4
  vCell : Outport  Port=5
  vParallelAssembly : Outport  Port=6
  wires:
  [vParallelAssembly2] -> vParallelAssemblyMux/2
  Module2_outputs/6 -> [vParallelAssembly2]
  [vCell2] -> vCellMux/2
  Module2_outputs/5 -> [vCell2]
  [socParallelAssembly2] -> socParallelAssemblyMux/2
  Module2_outputs/4 -> [socParallelAssembly2]
  [socCell2] -> socCellMux/2
  Module2_outputs/3 -> [socCell2]
  [numCyclesCell2] -> numCyclesCellMux/2
  Module2_outputs/2 -> [numCyclesCell2]
  [iCell2] -> iCellMux/2
  Module2_outputs/1 -> [iCell2]
  [vParallelAssembly1] -> vParallelAssemblyMux/1
  vParallelAssemblyMux/1 -> vParallelAssembly/1
  Module1_outputs/6 -> [vParallelAssembly1]
  [vCell1] -> vCellMux/1
  vCellMux/1 -> vCell/1
  Module1_outputs/5 -> [vCell1]
  [socParallelAssembly1] -> socParallelAssemblyMux/1
  socParallelAssemblyMux/1 -> socParallelAssembly/1
  Module1_outputs/4 -> [socParallelAssembly1]
  [socCell1] -> socCellMux/1
  socCellMux/1 -> socCell/1
  Module1_outputs/3 -> [socCell1]
  [numCyclesCell1] -> numCyclesCellMux/1
  numCyclesCellMux/1 -> numCyclesCell/1
  Module1_outputs/2 -> [numCyclesCell1]
  [iCell1] -> iCellMux/1
  iCellMux/1 -> iCell/1
  Module1_outputs/1 -> [iCell1]
  connections:
  Module2/RConn1 -- -/RConn1
  Module1/LConn1 -- +/RConn1
  Module2/LConn1 -- Module1/RConn1

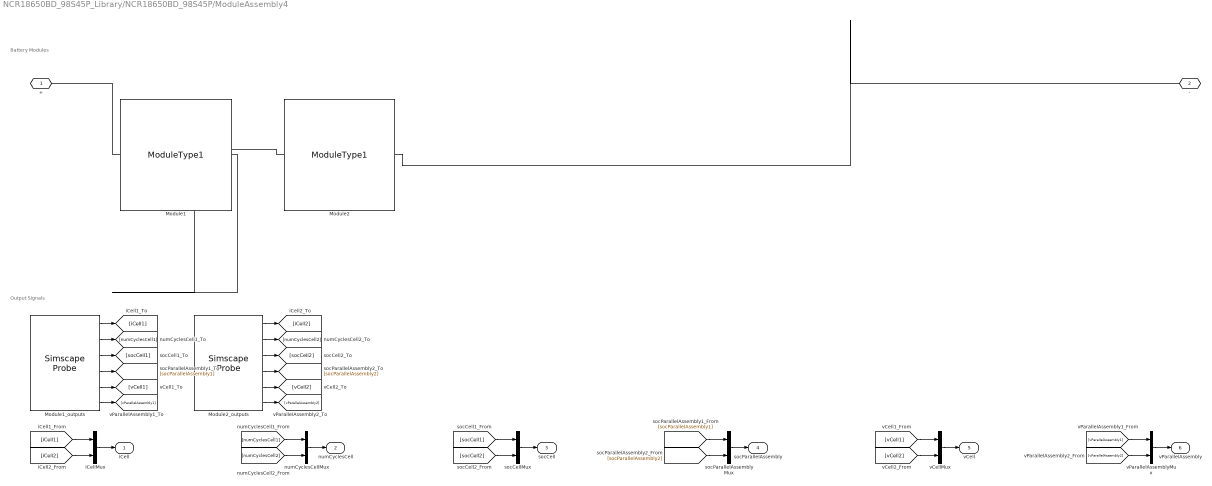
== system NCR18650BD_98S45P_Library/NCR18650BD_98S45P/ModuleAssembly4 ==
  note: Output Signals
  note: Battery Modules
  Module1 : NCR18650BD_98S45P_Library_lib/Modules/ModuleType1  SOC_vecCell=[0, .1, .25, .5, .75, .9, 1]  V0_vecCell=[3.5057, 3.566, 3.6337, 3.7127, 3.9259, 4.0777, 4.1928] V  V_rangeCell=[0, inf] V  R0_vecCell=[.0085, .0085, .0087, .0082, .0083, .0085, .0085] Ohm  AHCell=27 A*hr  extrapolation_optionCell=simscape.enum.extrapolation.nearest  P=45  S=7  iCell_specify=off  iCell_priority=None  iCell=0 A  iCell_nominal_specify=off  iCell_nominal_value=1  iCell_nominal_unit=A  vCell_specify=off  vCell_priority=None  vCell=0 V  vCell_nominal_specify=off  vCell_nominal_value=1  vCell_nominal_unit=V  socCell_specify=off  socCell_priority=High  socCell=1  socCell_nominal_specify=off  socCell_nominal_value=1  socCell_nominal_unit=1  numCyclesCell_specify=off  numCyclesCell_priority=High  numCyclesCell=0  numCyclesCell_nominal_specify=off  numCyclesCell_nominal_value=1  numCyclesCell_nominal_unit=1  vParallelAssembly_specify=off  vParallelAssembly_priority=None  vParallelAssembly=repmat(0, 7, 1) V  vParallelAssembly_nominal_specify=off  vParallelAssembly_nominal_value=1  vParallelAssembly_nominal_unit=V  socParallelAssembly_specify=off  socParallelAssembly_priority=None  socParallelAssembly=repmat(1, 7, 1)  socParallelAssembly_nominal_specify=off  socParallelAssembly_nominal_value=1  socParallelAssembly_nominal_unit=1
      settings: InternalSimscapePortConfiguration="{\"Bottom\":[{\"id\":\"n\",\"label\":\"-\",\"type\":\"foundation.electrical.electrical\"}],\"Left\":[],\"Right\":[],\"Top\":[{\"id\":\"p\",\"label\":\"+\",\"type\":\"foundation.electrical.electrical\"}]}"
  Module1_outputs : SimscapeProbe  BoundBlock=184  Variables="{\"iCell\":{\"Probing\":\"ON\"},\"numCyclesCell\":{\"Probing\":\"ON\"},\"socCell\":{\"Probing\":\"ON\"},\"socParallelAssembly\":{\"Probing\":\"ON\"},\"vCell\":{\"Probing\":\"ON\"},\"vParallelAssembly\":{\"Probing\":\"ON\"}}"
  Module2 : NCR18650BD_98S45P_Library_lib/Modules/ModuleType1  SOC_vecCell=[0, .1, .25, .5, .75, .9, 1]  V0_vecCell=[3.5057, 3.566, 3.6337, 3.7127, 3.9259, 4.0777, 4.1928] V  V_rangeCell=[0, inf] V  R0_vecCell=[.0085, .0085, .0087, .0082, .0083, .0085, .0085] Ohm  AHCell=27 A*hr  extrapolation_optionCell=simscape.enum.extrapolation.nearest  P=45  S=7  iCell_specify=off  iCell_priority=None  iCell=0 A  iCell_nominal_specify=off  iCell_nominal_value=1  iCell_nominal_unit=A  vCell_specify=off  vCell_priority=None  vCell=0 V  vCell_nominal_specify=off  vCell_nominal_value=1  vCell_nominal_unit=V  socCell_specify=off  socCell_priority=High  socCell=1  socCell_nominal_specify=off  socCell_nominal_value=1  socCell_nominal_unit=1  numCyclesCell_specify=off  numCyclesCell_priority=High  numCyclesCell=0  numCyclesCell_nominal_specify=off  numCyclesCell_nominal_value=1  numCyclesCell_nominal_unit=1  vParallelAssembly_specify=off  vParallelAssembly_priority=None  vParallelAssembly=repmat(0, 7, 1) V  vParallelAssembly_nominal_specify=off  vParallelAssembly_nominal_value=1  vParallelAssembly_nominal_unit=V  socParallelAssembly_specify=off  socParallelAssembly_priority=None  socParallelAssembly=repmat(1, 7, 1)  socParallelAssembly_nominal_specify=off  socParallelAssembly_nominal_value=1  socParallelAssembly_nominal_unit=1
      settings: InternalSimscapePortConfiguration="{\"Bottom\":[{\"id\":\"n\",\"label\":\"-\",\"type\":\"foundation.electrical.electrical\"}],\"Left\":[],\"Right\":[],\"Top\":[{\"id\":\"p\",\"label\":\"+\",\"type\":\"foundation.electrical.electrical\"}]}"
  Module2_outputs : SimscapeProbe  BoundBlock=186  Variables="{\"iCell\":{\"Probing\":\"ON\"},\"numCyclesCell\":{\"Probing\":\"ON\"},\"socCell\":{\"Probing\":\"ON\"},\"socParallelAssembly\":{\"Probing\":\"ON\"},\"vCell\":{\"Probing\":\"ON\"},\"vParallelAssembly\":{\"Probing\":\"ON\"}}"
  iCellMux : Mux  Inputs=2
  numCyclesCellMux : Mux  Inputs=2
  socCellMux : Mux  Inputs=2
  socParallelAssemblyMux : Mux  Inputs=2
  vCellMux : Mux  Inputs=2
  vParallelAssemblyMux : Mux  Inputs=2
  + : PMIOPort  Side=Left
  - : PMIOPort  Port=2  Side=Right
  iCell : Outport
  numCyclesCell : Outport  Port=2
  socCell : Outport  Port=3
  socParallelAssembly : Outport  Port=4
  vCell : Outport  Port=5
  vParallelAssembly : Outport  Port=6
  wires:
  [vParallelAssembly2] -> vParallelAssemblyMux/2
  Module2_outputs/6 -> [vParallelAssembly2]
  [vCell2] -> vCellMux/2
  Module2_outputs/5 -> [vCell2]
  [socParallelAssembly2] -> socParallelAssemblyMux/2
  Module2_outputs/4 -> [socParallelAssembly2]
  [socCell2] -> socCellMux/2
  Module2_outputs/3 -> [socCell2]
  [numCyclesCell2] -> numCyclesCellMux/2
  Module2_outputs/2 -> [numCyclesCell2]
  [iCell2] -> iCellMux/2
  Module2_outputs/1 -> [iCell2]
  [vParallelAssembly1] -> vParallelAssemblyMux/1
  vParallelAssemblyMux/1 -> vParallelAssembly/1
  Module1_outputs/6 -> [vParallelAssembly1]
  [vCell1] -> vCellMux/1
  vCellMux/1 -> vCell/1
  Module1_outputs/5 -> [vCell1]
  [socParallelAssembly1] -> socParallelAssemblyMux/1
  socParallelAssemblyMux/1 -> socParallelAssembly/1
  Module1_outputs/4 -> [socParallelAssembly1]
  [socCell1] -> socCellMux/1
  socCellMux/1 -> socCell/1
  Module1_outputs/3 -> [socCell1]
  [numCyclesCell1] -> numCyclesCellMux/1
  numCyclesCellMux/1 -> numCyclesCell/1
  Module1_outputs/2 -> [numCyclesCell1]
  [iCell1] -> iCellMux/1
  iCellMux/1 -> iCell/1
  Module1_outputs/1 -> [iCell1]
  connections:
  Module2/RConn1 -- -/RConn1
  Module1/LConn1 -- +/RConn1
  Module2/LConn1 -- Module1/RConn1

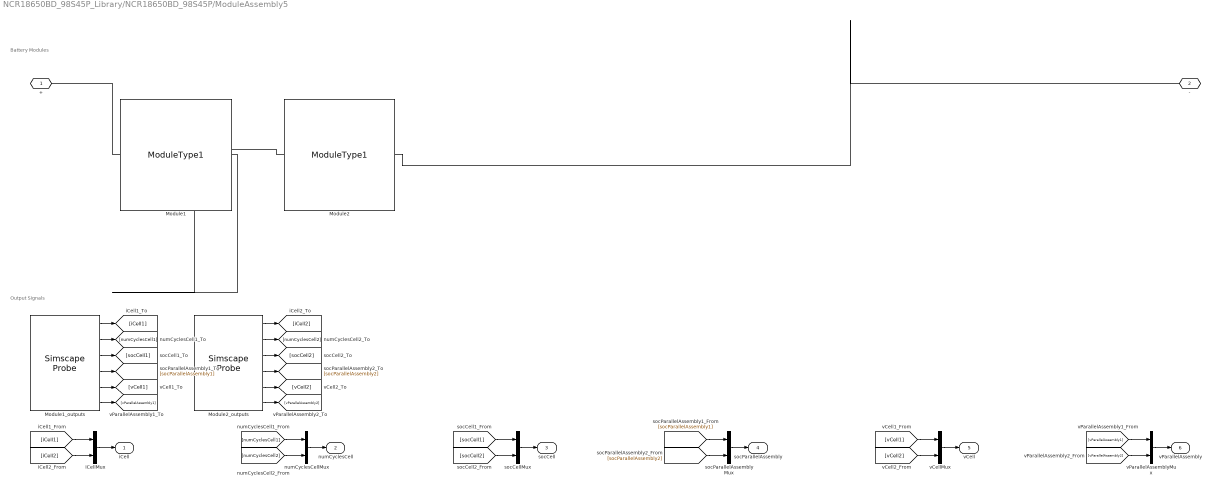
== system NCR18650BD_98S45P_Library/NCR18650BD_98S45P/ModuleAssembly5 ==
  note: Output Signals
  note: Battery Modules
  Module1 : NCR18650BD_98S45P_Library_lib/Modules/ModuleType1  SOC_vecCell=[0, .1, .25, .5, .75, .9, 1]  V0_vecCell=[3.5057, 3.566, 3.6337, 3.7127, 3.9259, 4.0777, 4.1928] V  V_rangeCell=[0, inf] V  R0_vecCell=[.0085, .0085, .0087, .0082, .0083, .0085, .0085] Ohm  AHCell=27 A*hr  extrapolation_optionCell=simscape.enum.extrapolation.nearest  P=45  S=7  iCell_specify=off  iCell_priority=None  iCell=0 A  iCell_nominal_specify=off  iCell_nominal_value=1  iCell_nominal_unit=A  vCell_specify=off  vCell_priority=None  vCell=0 V  vCell_nominal_specify=off  vCell_nominal_value=1  vCell_nominal_unit=V  socCell_specify=off  socCell_priority=High  socCell=1  socCell_nominal_specify=off  socCell_nominal_value=1  socCell_nominal_unit=1  numCyclesCell_specify=off  numCyclesCell_priority=High  numCyclesCell=0  numCyclesCell_nominal_specify=off  numCyclesCell_nominal_value=1  numCyclesCell_nominal_unit=1  vParallelAssembly_specify=off  vParallelAssembly_priority=None  vParallelAssembly=repmat(0, 7, 1) V  vParallelAssembly_nominal_specify=off  vParallelAssembly_nominal_value=1  vParallelAssembly_nominal_unit=V  socParallelAssembly_specify=off  socParallelAssembly_priority=None  socParallelAssembly=repmat(1, 7, 1)  socParallelAssembly_nominal_specify=off  socParallelAssembly_nominal_value=1  socParallelAssembly_nominal_unit=1
      settings: InternalSimscapePortConfiguration="{\"Bottom\":[{\"id\":\"n\",\"label\":\"-\",\"type\":\"foundation.electrical.electrical\"}],\"Left\":[],\"Right\":[],\"Top\":[{\"id\":\"p\",\"label\":\"+\",\"type\":\"foundation.electrical.electrical\"}]}"
  Module1_outputs : SimscapeProbe  BoundBlock=229  Variables="{\"iCell\":{\"Probing\":\"ON\"},\"numCyclesCell\":{\"Probing\":\"ON\"},\"socCell\":{\"Probing\":\"ON\"},\"socParallelAssembly\":{\"Probing\":\"ON\"},\"vCell\":{\"Probing\":\"ON\"},\"vParallelAssembly\":{\"Probing\":\"ON\"}}"
  Module2 : NCR18650BD_98S45P_Library_lib/Modules/ModuleType1  SOC_vecCell=[0, .1, .25, .5, .75, .9, 1]  V0_vecCell=[3.5057, 3.566, 3.6337, 3.7127, 3.9259, 4.0777, 4.1928] V  V_rangeCell=[0, inf] V  R0_vecCell=[.0085, .0085, .0087, .0082, .0083, .0085, .0085] Ohm  AHCell=27 A*hr  extrapolation_optionCell=simscape.enum.extrapolation.nearest  P=45  S=7  iCell_specify=off  iCell_priority=None  iCell=0 A  iCell_nominal_specify=off  iCell_nominal_value=1  iCell_nominal_unit=A  vCell_specify=off  vCell_priority=None  vCell=0 V  vCell_nominal_specify=off  vCell_nominal_value=1  vCell_nominal_unit=V  socCell_specify=off  socCell_priority=High  socCell=1  socCell_nominal_specify=off  socCell_nominal_value=1  socCell_nominal_unit=1  numCyclesCell_specify=off  numCyclesCell_priority=High  numCyclesCell=0  numCyclesCell_nominal_specify=off  numCyclesCell_nominal_value=1  numCyclesCell_nominal_unit=1  vParallelAssembly_specify=off  vParallelAssembly_priority=None  vParallelAssembly=repmat(0, 7, 1) V  vParallelAssembly_nominal_specify=off  vParallelAssembly_nominal_value=1  vParallelAssembly_nominal_unit=V  socParallelAssembly_specify=off  socParallelAssembly_priority=None  socParallelAssembly=repmat(1, 7, 1)  socParallelAssembly_nominal_specify=off  socParallelAssembly_nominal_value=1  socParallelAssembly_nominal_unit=1
      settings: InternalSimscapePortConfiguration="{\"Bottom\":[{\"id\":\"n\",\"label\":\"-\",\"type\":\"foundation.electrical.electrical\"}],\"Left\":[],\"Right\":[],\"Top\":[{\"id\":\"p\",\"label\":\"+\",\"type\":\"foundation.electrical.electrical\"}]}"
  Module2_outputs : SimscapeProbe  BoundBlock=231  Variables="{\"iCell\":{\"Probing\":\"ON\"},\"numCyclesCell\":{\"Probing\":\"ON\"},\"socCell\":{\"Probing\":\"ON\"},\"socParallelAssembly\":{\"Probing\":\"ON\"},\"vCell\":{\"Probing\":\"ON\"},\"vParallelAssembly\":{\"Probing\":\"ON\"}}"
  iCellMux : Mux  Inputs=2
  numCyclesCellMux : Mux  Inputs=2
  socCellMux : Mux  Inputs=2
  socParallelAssemblyMux : Mux  Inputs=2
  vCellMux : Mux  Inputs=2
  vParallelAssemblyMux : Mux  Inputs=2
  + : PMIOPort  Side=Left
  - : PMIOPort  Port=2  Side=Right
  iCell : Outport
  numCyclesCell : Outport  Port=2
  socCell : Outport  Port=3
  socParallelAssembly : Outport  Port=4
  vCell : Outport  Port=5
  vParallelAssembly : Outport  Port=6
  wires:
  [vParallelAssembly2] -> vParallelAssemblyMux/2
  Module2_outputs/6 -> [vParallelAssembly2]
  [vCell2] -> vCellMux/2
  Module2_outputs/5 -> [vCell2]
  [socParallelAssembly2] -> socParallelAssemblyMux/2
  Module2_outputs/4 -> [socParallelAssembly2]
  [socCell2] -> socCellMux/2
  Module2_outputs/3 -> [socCell2]
  [numCyclesCell2] -> numCyclesCellMux/2
  Module2_outputs/2 -> [numCyclesCell2]
  [iCell2] -> iCellMux/2
  Module2_outputs/1 -> [iCell2]
  [vParallelAssembly1] -> vParallelAssemblyMux/1
  vParallelAssemblyMux/1 -> vParallelAssembly/1
  Module1_outputs/6 -> [vParallelAssembly1]
  [vCell1] -> vCellMux/1
  vCellMux/1 -> vCell/1
  Module1_outputs/5 -> [vCell1]
  [socParallelAssembly1] -> socParallelAssemblyMux/1
  socParallelAssemblyMux/1 -> socParallelAssembly/1
  Module1_outputs/4 -> [socParallelAssembly1]
  [socCell1] -> socCellMux/1
  socCellMux/1 -> socCell/1
  Module1_outputs/3 -> [socCell1]
  [numCyclesCell1] -> numCyclesCellMux/1
  numCyclesCellMux/1 -> numCyclesCell/1
  Module1_outputs/2 -> [numCyclesCell1]
  [iCell1] -> iCellMux/1
  iCellMux/1 -> iCell/1
  Module1_outputs/1 -> [iCell1]
  connections:
  Module2/RConn1 -- -/RConn1
  Module1/LConn1 -- +/RConn1
  Module2/LConn1 -- Module1/RConn1
